simulink model "SNS_WinnerSlice_R8"  (R2025a)
settings: Solver=ode1  StartTime=0.0  StopTime=22  FixedStep=0.002  RelTol=1e-3
libraries: SNS_Library_R2025a x106, simulink x6
(part 2 of 2)

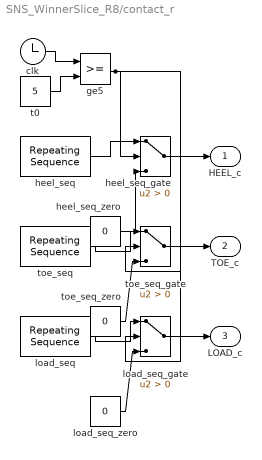
== system SNS_WinnerSlice_R8/contact_r ==
  clk : Clock
  ge5 : RelationalOperator  OutDataTypeStr=boolean  RndMeth=Simplest  InputSameDT=off
  heel_seq : simulink/Sources/Repeating Sequence  rep_seq_t=[0 0.008642 0.017284 0.025926 0.034568 0.04321 0.051852 0.060494 0.069136 0.077778 0.08642 0.095062 0.103704 0.112346 0.120988 0.12963 0.138272 0.146914 0.155556 0.164198 0.17284 0.181482 0.190124 0.198766 0.207408 0.21605 0.224692 0.233334 0.241976 0.250618 0.25926 0.267902 0.276544 0.285186 0.293828 0.30247 0.311112 0.319754 0.328396 0.337038 0.34568 0.354322 0.362964 0.371606 0.380248 0.38889 0.397532 0.406174 0.414816 0.423458 0.4321 0.440742 0.449384 0.458026 0.466668 0.47531 0.483952 0.492594 0.501236 0.509878 0.51852 0.527162 0.535804 0.544446 0.553088 0.56173 0.570372 0.579014 0.587656 0.596298 0.60494 0.613582 0.622224 0.630866 0.639508 0.64815 0.656792 0.665434 0.674076 0.682718 0.69136 0.700002 0.708644 0.717286 0.725928 0.73457 0.743212 0.751854 0.760496 0.769138 0.77778 0.786422 0.795064 0.803706 0.812348 0.82099 0.829632 0.838274 0.846916 0.855558 0.8642 0.872842 0.881484 0.890126 0.898768 0.90741 0.916052 0.924694 0.933336 0.941978 0.95062 0.959262 0.967904 0.976546 0.985188 0.99383 1.002472 1.011114 1.019756 1.028398 1.03704 1.045682 1.054324 1.062966 1.071608 1.08025 1.088892 1.097534 1.106176 1.114818 1.12346 1.132102 1.140744 1.149386 1.158028 1.16667 1.175312 1.183954 1.192596 1.201238 1.20988 1.218522 1.227164 1.235806 1.244448 1.25309 1.261732 1.270374 1.279016 1.287658 1.2963 1.304942 1.313584 1.322226 1.330868 1.33951 1.348152 1.356794 1.365436 1.374078 1.38272 1.391362 1.400004 1.408646 1.417288 1.42593 1.434572 1.443214 1.451856 1.460498 1.46914 1.477782 1.486424 1.495066 1.503708 1.51235 1.520992 1.529634 1.538276 1.546918 1.55556 1.564202 1.572844 1.581486 1.590128 1.59877 1.607412 1.616054 1.624696 1.633338 1.64198 1.650622 1.659264 1.667906 1.676548 1.68519 1.693832 1.702474 1.711116 1.719758 1.7284]  rep_seq_y=[0.817272721 1.460274974 2.104220735 2.749077948 2.935867053 2.911684299 2.88832321 2.86575587 2.843955308 2.822895471 2.802551192 2.782898157 2.763912881 2.745572674 2.727855618 2.710740541 2.69420699 2.678235204 2.662806098 2.647901231 2.633502793 2.619593576 2.606156956 2.593176878 2.580637828 2.568524822 2.556823384 2.54551953 2.53459975 2.524050996 2.513860661 2.504016566 2.494506948 2.485320441 2.476446067 2.467873221 2.459591658 2.45159148 2.443863127 2.436397364 2.429185267 2.422218218 2.41548789 2.408986242 2.402705502 2.361334428 2.308401593 2.255667905 2.203126599 2.150771137 2.098595205 2.046592703 1.994757738 1.943084618 1.891567844 1.840202104 1.788982265 1.73790337 1.686960632 1.636149422 1.585465273 1.552320378 1.519294055 1.486382276 1.453581149 1.420886915 1.38829594 1.355804718 1.323409858 1.291108087 1.258896241 1.226771266 1.194730209 1.162770219 1.130888541 1.099082516 1.067349572 1.035687226 1.00409308 0.972564816 0.941100196 0.909697057 0.878353311 0.847066939 0.815835992 0.784658587 0.753532904 0.722457186 0.691429736 0.660448914 0.629513134 0.598620868 0.567770635 0.536961009 0.506190609 0.475458103 0.444762203 0.414101665 0.383475288 0.352881911 0.322320413 0.29178971 0.261288757 0.230816542 0.200372089 0.169954455 0.139562729 0.10919603 0.078853508 0.048534341 0.018237736 0.017618066 0.017019451 0.016441175 0.015882547 0.0153429 0.014821589 0.014317991 0.013831503 0.013361546 0.012907556 0.012468991 0.012045328 0.011636059 0.011240697 0.010858768 0.010489816 0.010133399 0.009789093 0.009456486 0.00913518 0.00882479 0.008524947 0.008235292 0.007955479 0.007685173 0.007424051 0.007171801 0.006928122 0.006692723 0.006465322 0.006245648 0.006033437 0.005828437 -0.817272721 -0.789503958 -0.762678704 -0.736764901 -0.711731581 -0.687548826 -0.664187738 -0.641620397 -0.619819835 -0.598759998 -0.578415719 -0.558762684 -0.539777408 -0.521437201 -0.503720146 -0.486605069 -0.470071517 -0.454099732 -0.438670625 -0.423765759 -0.409367321 -0.395458103 -0.382021484 -0.369041405 -0.356502356 -0.344389349 -0.332687911 -0.321384057 -0.310464278 -0.299915524 -0.289725188 -0.279881094 -0.270371475 -0.261184968 -0.252310595 -0.243737749 -0.235456185 -0.227456008 -0.219727655 -0.212261891 -0.205049794 -0.198082745 -0.191352418 -0.184850769 -0.17857003 -0.172502693 -0.166641508 -0.160979471 -0.155509815 -0.150226003 -0.145121721 -0.140190869 -0.135427555 -0.130826085 -0.126380961 -0.122086871 -0.117938682]
  heel_seq_gate : Switch  Criteria=u2 > Threshold  SaturateOnIntegerOverflow=off  InputSameDT=off
  heel_seq_zero : Constant  Value=0
  load_seq : simulink/Sources/Repeating Sequence  rep_seq_t=[0 0.008642 0.017284 0.025926 0.034568 0.04321 0.051852 0.060494 0.069136 0.077778 0.08642 0.095062 0.103704 0.112346 0.120988 0.12963 0.138272 0.146914 0.155556 0.164198 0.17284 0.181482 0.190124 0.198766 0.207408 0.21605 0.224692 0.233334 0.241976 0.250618 0.25926 0.267902 0.276544 0.285186 0.293828 0.30247 0.311112 0.319754 0.328396 0.337038 0.34568 0.354322 0.362964 0.371606 0.380248 0.38889 0.397532 0.406174 0.414816 0.423458 0.4321 0.440742 0.449384 0.458026 0.466668 0.47531 0.483952 0.492594 0.501236 0.509878 0.51852 0.527162 0.535804 0.544446 0.553088 0.56173 0.570372 0.579014 0.587656 0.596298 0.60494 0.613582 0.622224 0.630866 0.639508 0.64815 0.656792 0.665434 0.674076 0.682718 0.69136 0.700002 0.708644 0.717286 0.725928 0.73457 0.743212 0.751854 0.760496 0.769138 0.77778 0.786422 0.795064 0.803706 0.812348 0.82099 0.829632 0.838274 0.846916 0.855558 0.8642 0.872842 0.881484 0.890126 0.898768 0.90741 0.916052 0.924694 0.933336 0.941978 0.95062 0.959262 0.967904 0.976546 0.985188 0.99383 1.002472 1.011114 1.019756 1.028398 1.03704 1.045682 1.054324 1.062966 1.071608 1.08025 1.088892 1.097534 1.106176 1.114818 1.12346 1.132102 1.140744 1.149386 1.158028 1.16667 1.175312 1.183954 1.192596 1.201238 1.20988 1.218522 1.227164 1.235806 1.244448 1.25309 1.261732 1.270374 1.279016 1.287658 1.2963 1.304942 1.313584 1.322226 1.330868 1.33951 1.348152 1.356794 1.365436 1.374078 1.38272 1.391362 1.400004 1.408646 1.417288 1.42593 1.434572 1.443214 1.451856 1.460498 1.46914 1.477782 1.486424 1.495066 1.503708 1.51235 1.520992 1.529634 1.538276 1.546918 1.55556 1.564202 1.572844 1.581486 1.590128 1.59877 1.607412 1.616054 1.624696 1.633338 1.64198 1.650622 1.659264 1.667906 1.676548 1.68519 1.693832 1.702474 1.711116 1.719758 1.7284]  rep_seq_y=[0 0.082391175 0.164782351 0.247173526 0.329564702 0.411955877 0.468328786 0.468328786 0.468328786 0.468328786 0.468328786 0.465437868 0.459656031 0.453874194 0.448092357 0.442310521 0.436528684 0.430746847 0.42496501 0.419183173 0.413401336 0.407619499 0.401837662 0.396055826 0.390273989 0.384492152 0.378710315 0.372928478 0.367146641 0.361364804 0.355582968 0.349801131 0.344019294 0.338237457 0.33245562 0.326673783 0.320891946 0.315110109 0.309328273 0.303546436 0.297764599 0.291982762 0.286200925 0.280419088 0.274637251 0.268855414 0.263073578 0.257291741 0.251509904 0.245728067 0.23994623 0.234164393 0.228382556 0.22260072 0.216818883 0.211037046 0.205255209 0.199473372 0.193691535 0.187909698 0.182127861 0.184209323 0.186290784 0.188372245 0.190453707 0.192535168 0.194616629 0.19669809 0.198779552 0.200861013 0.202942474 0.205023935 0.207105397 0.209186858 0.211268319 0.213349781 0.215431242 0.217512703 0.219594164 0.221675626 0.223757087 0.225838548 0.227920009 0.230001471 0.232082932 0.234164393 0.236245855 0.238327316 0.240408777 0.242490238 0.2445717 0.246653161 0.248734622 0.250816083 0.252897545 0.254979006 0.257060467 0.259141929 0.26122339 0.263304851 0.265386312 0.267467774 0.269549235 0.271630696 0.273712157 0.275793619 0.27787508 0.279956541 0.282038003 0.284119464 0.286200925 0.286200925 0.286200925 0.286200925 0.286200925 0.286200925 0.286200925 0.286200925 0.286200925 0.286200925 0.286200925 0.286200925 0.286200925 0.286200925 0.286200925 0.299210058 0.312219191 0.325228324 0.338237457 0.35124659 0.364255723 0.377264856 0.390273989 0.403283122 0.416292255 0.429301388 0.442310521 0.455319654 0.468328786 0.468328786 0.468328786 0.370760289 0.247173526 0.123586763 0 0 0 0 0 0 0 0 0 0 0 0 0 0 0 0 0 0 0 0 0 0 0 0 0 0 0 0 0 0 0 0 0 0 0 0 0 0 0 0 0 0 0 0 0 0 0 0 0 0 0 0 0 0 0 0 0]
  load_seq_gate : Switch  Criteria=u2 > Threshold  SaturateOnIntegerOverflow=off  InputSameDT=off
  load_seq_zero : Constant  Value=0
  t0 : Constant  Value=5
  toe_seq : simulink/Sources/Repeating Sequence  rep_seq_t=[0 0.008642 0.017284 0.025926 0.034568 0.04321 0.051852 0.060494 0.069136 0.077778 0.08642 0.095062 0.103704 0.112346 0.120988 0.12963 0.138272 0.146914 0.155556 0.164198 0.17284 0.181482 0.190124 0.198766 0.207408 0.21605 0.224692 0.233334 0.241976 0.250618 0.25926 0.267902 0.276544 0.285186 0.293828 0.30247 0.311112 0.319754 0.328396 0.337038 0.34568 0.354322 0.362964 0.371606 0.380248 0.38889 0.397532 0.406174 0.414816 0.423458 0.4321 0.440742 0.449384 0.458026 0.466668 0.47531 0.483952 0.492594 0.501236 0.509878 0.51852 0.527162 0.535804 0.544446 0.553088 0.56173 0.570372 0.579014 0.587656 0.596298 0.60494 0.613582 0.622224 0.630866 0.639508 0.64815 0.656792 0.665434 0.674076 0.682718 0.69136 0.700002 0.708644 0.717286 0.725928 0.73457 0.743212 0.751854 0.760496 0.769138 0.77778 0.786422 0.795064 0.803706 0.812348 0.82099 0.829632 0.838274 0.846916 0.855558 0.8642 0.872842 0.881484 0.890126 0.898768 0.90741 0.916052 0.924694 0.933336 0.941978 0.95062 0.959262 0.967904 0.976546 0.985188 0.99383 1.002472 1.011114 1.019756 1.028398 1.03704 1.045682 1.054324 1.062966 1.071608 1.08025 1.088892 1.097534 1.106176 1.114818 1.12346 1.132102 1.140744 1.149386 1.158028 1.16667 1.175312 1.183954 1.192596 1.201238 1.20988 1.218522 1.227164 1.235806 1.244448 1.25309 1.261732 1.270374 1.279016 1.287658 1.2963 1.304942 1.313584 1.322226 1.330868 1.33951 1.348152 1.356794 1.365436 1.374078 1.38272 1.391362 1.400004 1.408646 1.417288 1.42593 1.434572 1.443214 1.451856 1.460498 1.46914 1.477782 1.486424 1.495066 1.503708 1.51235 1.520992 1.529634 1.538276 1.546918 1.55556 1.564202 1.572844 1.581486 1.590128 1.59877 1.607412 1.616054 1.624696 1.633338 1.64198 1.650622 1.659264 1.667906 1.676548 1.68519 1.693832 1.702474 1.711116 1.719758 1.7284]  rep_seq_y=[0.817272721 0.789503958 0.762678704 0.736764901 0.711731581 0.687548826 0.664187738 0.641620397 0.619819835 0.598759998 0.578415719 0.558762684 0.539777408 0.521437201 0.503720146 0.486605069 0.470071517 0.454099732 0.438670625 0.423765759 0.409367321 0.395458103 0.382021484 0.369041405 0.356502356 0.344389349 0.332687911 0.321384057 0.310464278 0.299915524 0.289725188 0.279881094 0.270371475 0.261184968 0.252310595 0.243737749 0.235456185 0.227456008 0.219727655 0.212261891 0.205049794 0.198082745 0.191352418 0.184850769 0.17857003 0.172502693 0.166641508 0.160979471 0.155509815 0.150226003 0.145121721 0.140190869 0.135427555 0.130826085 0.126380961 0.122086871 0.117938682 0.113931438 0.110060349 0.10632079 0.102708291 0.107138637 0.111687555 0.116351017 0.121125131 0.126006138 0.130990405 0.136074423 0.141254805 0.146528274 0.15189167 0.157341935 0.162876119 0.16849137 0.174184934 0.179954149 0.185796446 0.191709341 0.197690436 0.203737413 0.209848034 0.216020137 0.222251631 0.2285405 0.234884794 0.24128263 0.247732188 0.254231712 0.260779503 0.267373921 0.274013383 0.280696357 0.287421366 0.294186981 0.300991822 0.307834557 0.314713897 0.321628601 0.328577464 0.335559328 0.342573071 0.34961761 0.356691897 0.363794924 0.370925712 0.378083319 0.385266834 0.392475375 0.399708094 0.406964168 0.414242805 0.413623135 0.413024519 0.412446243 0.411887616 0.411347969 0.410826658 0.41032306 0.409836572 0.409366614 0.408912624 0.40847406 0.408050396 0.407641128 0.407245766 0.424864067 0.442495345 0.460139159 0.477795084 0.495462707 0.513141631 0.530831472 0.548531859 0.548242204 0.547962391 0.547692085 0.547430963 0.547178713 0.546935034 0.546699635 0.546472234 0.519252214 0.348037815 0.176830626 -0.817272721 -0.789503958 -0.762678704 -0.736764901 -0.711731581 -0.687548826 -0.664187738 -0.641620397 -0.619819835 -0.598759998 -0.578415719 -0.558762684 -0.539777408 -0.521437201 -0.503720146 -0.486605069 -0.470071517 -0.454099732 -0.438670625 -0.423765759 -0.409367321 -0.395458103 -0.382021484 -0.369041405 -0.356502356 -0.344389349 -0.332687911 -0.321384057 -0.310464278 -0.299915524 -0.289725188 -0.279881094 -0.270371475 -0.261184968 -0.252310595 -0.243737749 -0.235456185 -0.227456008 -0.219727655 -0.212261891 -0.205049794 -0.198082745 -0.191352418 -0.184850769 -0.17857003 -0.172502693 -0.166641508 -0.160979471 -0.155509815 -0.150226003 -0.145121721 -0.140190869 -0.135427555 -0.130826085 -0.126380961 -0.122086871 -0.117938682]
  toe_seq_gate : Switch  Criteria=u2 > Threshold  SaturateOnIntegerOverflow=off  InputSameDT=off
  toe_seq_zero : Constant  Value=0
  HEEL_c : Outport
  TOE_c : Outport  Port=2
  LOAD_c : Outport  Port=3
  wires:
  clk/1 -> ge5/1
  t0/1 -> ge5/2
  heel_seq/1 -> heel_seq_gate/1
  ge5/1 -> heel_seq_gate/2, toe_seq_gate/2, load_seq_gate/2
  heel_seq_zero/1 -> heel_seq_gate/3
  heel_seq_gate/1 -> HEEL_c/1
  toe_seq/1 -> toe_seq_gate/1
  toe_seq_zero/1 -> toe_seq_gate/3
  toe_seq_gate/1 -> TOE_c/1
  load_seq/1 -> load_seq_gate/1
  load_seq_zero/1 -> load_seq_gate/3
  load_seq_gate/1 -> LOAD_c/1
